simulink model "L2_scheme"  (R2019b)
settings: Solver=VariableStepAuto  StartTime=0.0  StopTime=10  RelTol=1e-3
settings Model: Creator=anton  LastModifiedBy=anton

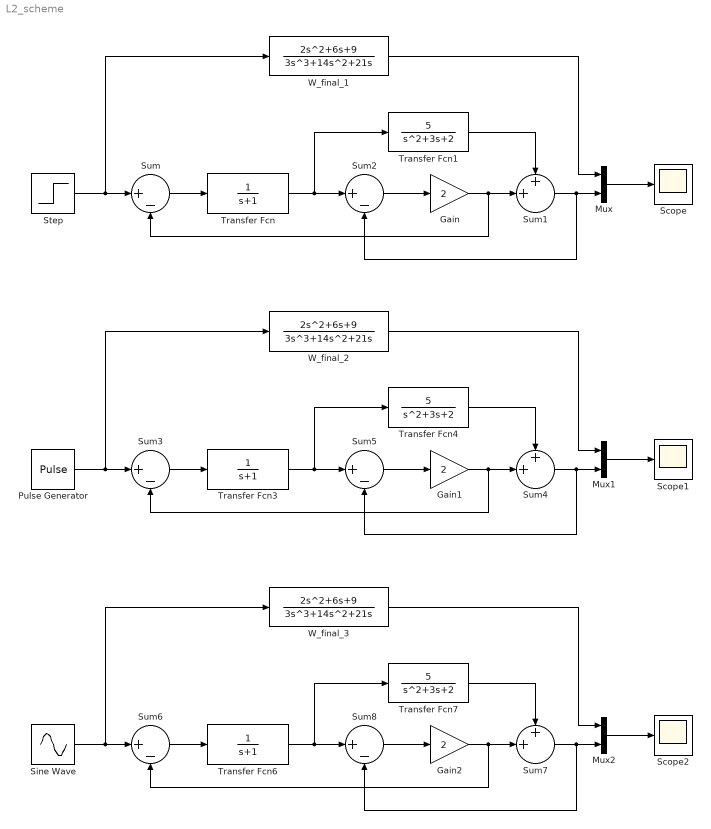
== system L2_scheme ==
  Gain : Gain  Gain=2
  Gain1 : Gain  Gain=2
  Gain2 : Gain  Gain=2
  Mux : Mux  Inputs=2
  Mux1 : Mux  Inputs=2
  Mux2 : Mux  Inputs=2
  Pulse Generator : DiscretePulseGenerator  PulseType=Time based  Period=5  PulseWidth=5
  Scope : Scope
  Scope1 : Scope
  Scope2 : Scope
  Sine Wave : Sin  SampleTime=0
  Step : Step  Time=5  After=5  SampleTime=0
  Sum{,2..3,5..6,8} (6 alike) : Sum  Inputs=|+-
  Sum1 : Sum  Inputs=++|
  Sum4 : Sum  Inputs=++|
  Sum7 : Sum  Inputs=++|
  Transfer Fcn : TransferFcn  Denominator=[1 1]
  Transfer Fcn1 : TransferFcn  Numerator=[5]  Denominator=[1 3 2]
  Transfer Fcn3 : TransferFcn  Denominator=[1 1]
  Transfer Fcn4 : TransferFcn  Numerator=[5]  Denominator=[1 3 2]
  Transfer Fcn6 : TransferFcn  Denominator=[1 1]
  Transfer Fcn7 : TransferFcn  Numerator=[5]  Denominator=[1 3 2]
  W_final_1 : TransferFcn  Numerator=[2 6 9]  Denominator=[3 14 21 0]
  W_final_2 : TransferFcn  Numerator=[2 6 9]  Denominator=[3 14 21 0]
  W_final_3 : TransferFcn  Numerator=[2 6 9]  Denominator=[3 14 21 0]
  wires:
  Sum/1 -> Transfer Fcn/1
  Transfer Fcn/1 -> Transfer Fcn1/1, Sum2/1
  Sum2/1 -> Gain/1
  Gain/1 -> Sum/2, Sum1/2
  Transfer Fcn1/1 -> Sum1/1
  Sum1/1 -> Sum2/2, Mux/2
  Step/1 -> W_final_1/1, Sum/1
  Mux/1 -> Scope/1
  W_final_1/1 -> Mux/1
  Transfer Fcn4/1 -> Sum4/1
  Sum3/1 -> Transfer Fcn3/1
  Sum4/1 -> Sum5/2, Mux1/2
  Mux1/1 -> Scope1/1
  Pulse Generator/1 -> W_final_2/1, Sum3/1
  Gain1/1 -> Sum3/2, Sum4/2
  Transfer Fcn3/1 -> Transfer Fcn4/1, Sum5/1
  W_final_2/1 -> Mux1/1
  Sum5/1 -> Gain1/1
  Transfer Fcn6/1 -> Transfer Fcn7/1, Sum8/1
  Sum8/1 -> Gain2/1
  Sine Wave/1 -> W_final_3/1, Sum6/1
  W_final_3/1 -> Mux2/1
  Sum6/1 -> Transfer Fcn6/1
  Sum7/1 -> Sum8/2, Mux2/2
  Mux2/1 -> Scope2/1
  Gain2/1 -> Sum6/2, Sum7/2
  Transfer Fcn7/1 -> Sum7/1
